simulink model "TESTLon"  (R2021b)
settings: Solver=VariableStepAuto  StartTime=0.0  StopTime=10.0  RelTol=1e-3
libraries: LPVBlockLibrary x2
settings Model: Creator=jihoo  LastModifiedBy=jihoo

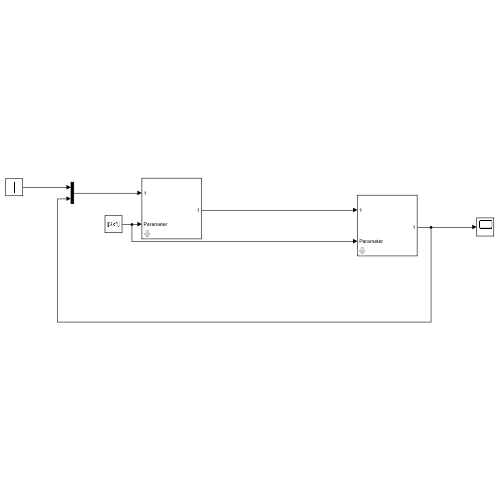
[thumbnail: Simulink's stored preview of the top-level diagram]
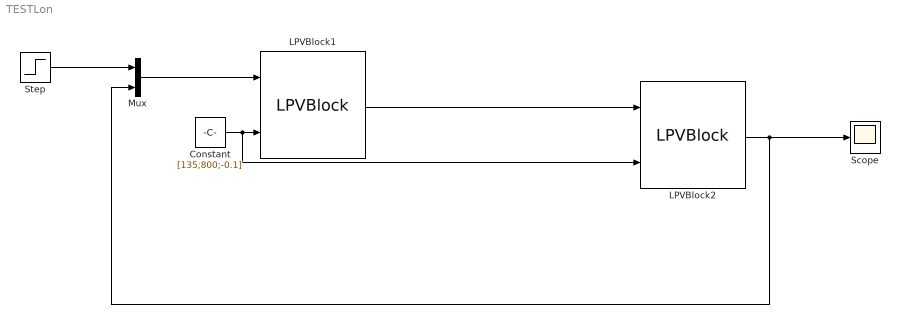
== system TESTLon ==
  Constant : Constant  Value=[135;800;-0.1]
  LPVBlock1 : LPVBlockLibrary/LPVBlock  sys=K_lon_lpv  plist={'rho1_tas_param';'rho2_alt_param';'rho3_mor_param'}  x0=0
      settings: SourceProductName=LPVTools Blocks
  LPVBlock2 : LPVBlockLibrary/LPVBlock  sys=P_lon  plist={'rho1_tas_param';'rho2_alt_param';'rho3_mor_param'}  x0=0
      settings: SourceProductName=LPVTools Blocks
  Mux : Mux  Inputs=2
  Scope : Scope
  Step : Step  SampleTime=0
  wires:
  LPVBlock1/1 -> LPVBlock2/1
  Constant/1 -> LPVBlock2/2, LPVBlock1/2
  LPVBlock2/1 -> Scope/1, Mux/2
  Mux/1 -> LPVBlock1/1
  Step/1 -> Mux/1
